simulink model "orig_exp_first_order"  (R2023a)
settings: Solver=ode4  StartTime=0.0  StopTime=10  FixedStep=0.0001  RelTol=1e-3
settings Model: Creator=Anonymous  LastModifiedBy=Anonymous

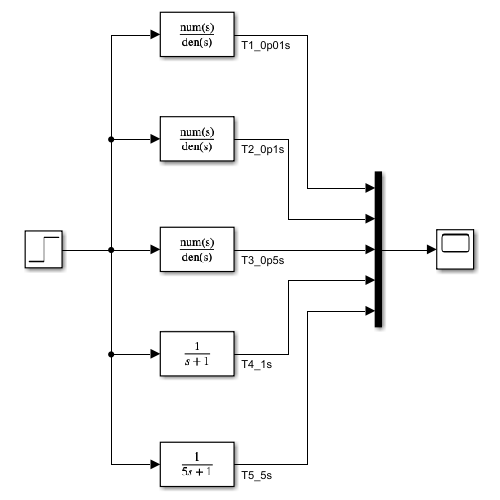
[thumbnail: Simulink's stored preview of the top-level diagram]
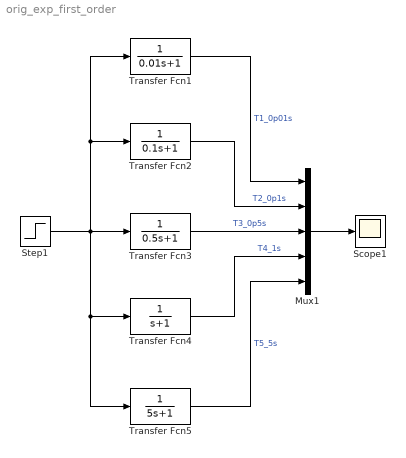
== system orig_exp_first_order ==
  Mux1 : Mux  Inputs=5
  Scope1 : Scope
  Step1 : Step  SampleTime=0
  Transfer Fcn1 : TransferFcn  Numerator=1  Denominator=[0.01 1]
  Transfer Fcn2 : TransferFcn  Numerator=1  Denominator=[0.1 1]
  Transfer Fcn3 : TransferFcn  Numerator=1  Denominator=[0.5 1]
  Transfer Fcn4 : TransferFcn  Numerator=1  Denominator=[1 1]
  Transfer Fcn5 : TransferFcn  Numerator=1  Denominator=[5 1]
  wires:
  Mux1/1 -> Scope1/1
  Transfer Fcn5/1 -> Mux1/5  "T5_5s"
  Transfer Fcn4/1 -> Mux1/4  "T4_1s"
  Transfer Fcn3/1 -> Mux1/3  "T3_0p5s"
  Transfer Fcn2/1 -> Mux1/2  "T2_0p1s"
  Transfer Fcn1/1 -> Mux1/1  "T1_0p01s"
  Step1/1 -> Transfer Fcn5/1, Transfer Fcn4/1, Transfer Fcn2/1, Transfer Fcn1/1, Transfer Fcn3/1
